simulink model "Porsche930Turbo_Model_V0"  (R2025b)
settings: Solver=ode3  StartTime=0.0  StopTime=1800  FixedStep=0.005  MaxStep=0.01  RelTol=1e-3
values from neighbouring files (symbols this model uses):
  a_front = (1 - CoG_front) * wb    (= 1.32912)    [Main.m]
  af = 1.77    [Main.m]
  bsfc = 395    [Main.m]
  cd = 0.39    [Main.m]
  crr = 0.015    [Main.m]
  distance_imola = s_track    [Main.m]
  eta_gb = 0.95    [Main.m]
  gear_numbers = [1, 2, 3, 4]    [Main.m]
  gear_ratios = [2.25, 1.30, 0.89, 0.625]    [Main.m]
  gear_shift_tbl = [1, 2, 3, 4]    [Main.m]
  grade_imola = grade_track    [Main.m]
  kt = 1.65    [Main.m]
  m_eq = mg + (J_wheels / rw^2) + (J_drivetrain * i_avg^2 / rw^2)    [Main.m]
  mg = mc + (mh * np) + mp_hybrid    (= 1492.5)    [Main.m]
  mu_road = 0.9    [Main.m]
  n_ice = 0:dn:nd    [Main.m]
  ne_em = 0:dn:nemax_em    [Main.m]
  nparallel = 2    [Main.m]
  nseries = 96    [Main.m]
  rho_fuel = 0.75    [Main.m]
  ro = 1.204    [Main.m]
  rt = 4.222    [Main.m]
  rw = (dw * 25.4 / 2 + wt * art / 100) * 1e-3    (= 0.31345)    [Main.m]
  t_ice = zeros(size(n_ice))    [Main.m]
  t_roma_san_basilio = [0 1 2 3 4 5 6 7 8 9 10 11 ... (522 elements, 522x1)]    [ECE_EUDC_Artemis_Bologna_Roma_WLTC_EE_bus.mat]
  tau_turbo = 0.6    [Main.m]
  te_em = zeros(size(ne_em))    [Main.m]
  te_em_peak = zeros(size(ne_em))    [Main.m]
  temax_em = 230    [Main.m]
  tmax_ice = 412    [Main.m]
  track_length = 4909    [Main.m]
  v_cutoff_bp = [0, 0.5, 1.4, 50]    [Main.m]
  v_cutoff_tbl = [0, 0,   1,   1 ]    [Main.m]
  v_ref_imola = v_track_ms    [Main.m]
  v_shift_bp = [0, 18, 33, 48]    [Main.m]
  v_shift_bp_EMODE = [0, 5, 22, 35]    [Main.m]
  vkm_roma_san_basilio = [28.8 30.9 32.4 34.2 35.3 35.6 34.8 33.8 32.2 30.5 29.1 27.9 ... (522 elements, 522x1)]    [ECE_EUDC_Artemis_Bologna_Roma_WLTC_EE_bus.mat]
  wb = 2.272    [Main.m]
undefined symbols (not defined in the file or in its folder): SoC_Per
libraries: simulink x58
(part 3 of 5)

== system Porsche930Turbo_Model_V0/Battery Pack/Subsystem/SOC Evalutation ==
  iB [A] : Inport
  SOH [%] : Inport  Port=2
  Battery Efficency [%] : Constant  Value=BattEff  OutDataTypeStr=single
  Compare To Constant : simulink/Logic and Bit Operations/Compare To Constant  relop=>=  const=0  OutDataTypeStr=boolean
  Constant : Constant  OutDataTypeStr=single
  Constant1 : Constant  OutDataTypeStr=single
  Cp(SOH) : Fcn  Expr=u(1)*u(4)^2 + u(2)*u(4) + u(3)
  Cp_coeff : Constant  Value=Cp  OutDataTypeStr=single
  Display{,1..3} (4 alike) : Display
  Divide : Product  Inputs=*/
  Gain : Gain  Gain=100
  Gain1 : Gain  Gain=1/100
  Gain2 : Gain  Gain=1/100
  Gain3 : Gain  Gain=1/100
  Memory : Memory  InitialCondition=InitialSOC
  Mux6 : Mux  Inputs=2
  Product : Product  OutDataTypeStr=single
  Product1 : Product
  Saturation1 : Saturate  UpperLimit=0.999  LowerLimit=0.001
  Saturation2 : Saturate  UpperLimit=0.999  LowerLimit=0.001
  Sum : Sum  Inputs=+-|  OutDataTypeStr=single
  Switch : Switch  Criteria=u2 > Threshold  SaturateOnIntegerOverflow=off  InputSameDT=off
  "[As] -> [Ah]" : Gain  Gain=1/3600
  dt [s] : SampleTimeMath  TsampMathOp=Ts Only
  SOC [%] : Outport
  wires:
  Cp_coeff/1 -> Display2/1, Mux6/1
  Mux6/1 -> Cp(SOH)/1
  Constant/1 -> dt [s]/1
  dt [s]/1 -> Display/1, Product/1
  Cp(SOH)/1 -> Display3/1, Divide/2
  Gain/1 -> Memory/1, Display1/1, SOC [%]/1
  Saturation1/1 -> Sum/1
  Sum/1 -> Saturation2/1
  Memory/1 -> Gain1/1
  Gain1/1 -> Saturation1/1
  iB [A]/1 -> Compare To Constant/1, Product/2
  "[As] -> [Ah]"/1 -> Sum/2
  Divide/1 -> "[As] -> [Ah]"/1
  Product1/1 -> Divide/1
  Product/1 -> Product1/1
  Switch/1 -> Product1/2
  Constant1/1 -> Switch/1
  Compare To Constant/1 -> Switch/2
  Battery Efficency [%]/1 -> Gain2/1
  Gain2/1 -> Switch/3
  SOH [%]/1 -> Gain3/1
  Gain3/1 -> Mux6/2
  Saturation2/1 -> Gain/1

== system Porsche930Turbo_Model_V0/Battery Pack/Subsystem/Thermal Model ==
  PowrLoss(t) [W] : Inport
  TAmb [°C] : Inport  Port=2
  Compare To Constant : simulink/Logic and Bit Operations/Compare To Constant  relop===  const=2  OutDataTypeStr=boolean
  Compare To Constant1 : simulink/Logic and Bit Operations/Compare To Constant  relop===  const=3  OutDataTypeStr=boolean
  Compare To Constant2 : simulink/Logic and Bit Operations/Compare To Constant  relop===  const=1  OutDataTypeStr=boolean
  Constant : Constant  OutDataTypeStr=single
  Constant1 : Constant  Value=R2Therml  OutDataTypeStr=single
  Constant2 : Constant  Value=R1Therml  OutDataTypeStr=single
  Constant3 : Constant  Value=R3Therml  OutDataTypeStr=single
  Constant4 : Constant  Value=C1Thermal  OutDataTypeStr=single
  Constant5 : Constant  Value=C2Thermal  OutDataTypeStr=single
  Delay : Delay  DelayLength=1  InitialConditionSource=Input port
      settings: InputPortMap=u0,p4
  Delay One Step : Delay  DelayLength=1  InitialCondition=25
  Display Temp : Constant  Value=TRoom  OutDataTypeStr=single
  Merge : Merge  Inputs=3
  Mux : Mux  Inputs=5
  Reference : Constant  Value=ThermReff  OutDataTypeStr=single
  Subsystem : Subsystem
  Subsystem1 : Subsystem
  Subsystem2 : Subsystem
  Sum : Sum  Inputs=|+-
  Switch1 : Switch  Criteria=u2 > Threshold  Threshold=0.5  SaturateOnIntegerOverflow=off  InputSameDT=off
  T_amb : Constant  Value=25
  Thermal Model Selector : Constant  Value=ThermalModelType  OutDataTypeStr=single
  air cooling : MATLAB Function  TreatAsAtomicUnit=on
  dt [s] : SampleTimeMath  TsampMathOp=Ts Only
  CellT [°C] : Outport
  wires:
  Mux/1 -> Subsystem/3(ModelThermalParam), Subsystem1/3(ModelThermalParam)
  Constant2/1 -> Mux/1
  Constant1/1 -> Mux/2
  Constant3/1 -> Mux/3
  Constant4/1 -> Mux/4
  Constant5/1 -> Mux/5
  dt [s]/1 -> Subsystem/4(dt), Subsystem1/4(dt)
  Constant/1 -> dt [s]/1
  Thermal Model Selector/1 -> Compare To Constant/1, Compare To Constant1/1, Compare To Constant2/1
  Compare To Constant/1 -> Subsystem/Enable
  Compare To Constant1/1 -> Subsystem1/Enable
  Subsystem/1(CellT [°C]) -> Merge/2
  Subsystem1/1(CellT [°C]) -> Merge/3
  Merge/1 -> Delay/1
  Delay/1 -> [cellT], CellT [°C]/1
  Display Temp/1 -> Switch1/1
  Reference/1 -> Switch1/2
  TAmb [°C]/1 -> Switch1/3
  Switch1/1 -> Subsystem2/1(TAmb [°C]), Subsystem/1(TAmb [°C]), Delay/2, Subsystem1/1(TAmb [°C])
  Compare To Constant2/1 -> Subsystem2/Enable
  Subsystem2/1(CellT [°C]) -> Merge/1
  [cellT] -> Delay One Step/1
  PowrLoss(t) [W]/1 -> Sum/1
  Sum/1 -> Subsystem1/2(InPower [W]), Subsystem/2(InPower [W])
  [speed] -> air cooling/1(v_car)
  Delay One Step/1 -> air cooling/2(T_cell)
  T_amb/1 -> air cooling/3(T_amb)
  air cooling/1(Q_cool) -> Sum/2

== system Porsche930Turbo_Model_V0/Battery Pack/Subsystem/Vb Evaluation ==
  iB(t) [A] : Inport
  SOC [%] : Inport  Port=2
  SOH [%] : Inport  Port=3
  TCell [°C] : Inport  Port=4
  Gain : Gain  Gain=1/100  OutDataTypeStr=single
  Gain1 : Gain  Gain=1/100
  Product : Product  OutDataTypeStr=single
  Product1 : Product  OutDataTypeStr=single
  R0 : Subsystem
  R0 * iB^2 : Product  OutDataTypeStr=single
  R1 : Subsystem
  Saturation : Saturate  UpperLimit=inf  LowerLimit=0
  Scope : Scope  NumInputPorts=3
      settings: ActiveDisplayYMinimum=-1  ActiveDisplayYMaximum=1  DataLoggingVariableName=ScopeData38
  Sum : Sum  Inputs=+--  OutDataTypeStr=single
  Sum1 : Sum  OutDataTypeStr=single
  VOC : Subsystem
  Vc (t) : Subsystem
  tau1 : Subsystem
  vB(t) [V] : Outport
  PowrLoss(t) [W] : Outport  Port=2
  wires:
  SOC [%]/1 -> Gain/1
  Gain/1 -> tau1/1(SOC [ ]), R1/1(SOC [ ]), R0/1(SOC [ ]), VOC/1(SOC [ ])
  SOH [%]/1 -> Gain1/1
  Gain1/1 -> R0/3(SOH [ ])
  TCell [°C]/1 -> R1/2(TCell [°C]), R0/2(TCell [°C])
  iB(t) [A]/1 -> Saturation/1
  R1/1(R1 [Ohm]) -> Vc (t)/2(R1 [Ohm])
  tau1/1(tau1 [s]) -> Vc (t)/3(tau1 [s])
  VOC/1(VOC [V]) -> Scope/1, Sum/1
  Product/1 -> Scope/2, Sum/2
  R0/1(R0 [Ohm]) -> R0 * iB^2/2, Product/2
  Vc (t)/1(Vc(t) [V]) -> Sum/3, Scope/3
  Sum/1 -> vB(t) [V]/1
  R0 * iB^2/1 -> Sum1/1
  Product1/1 -> R0 * iB^2/1
  Vc (t)/2(PowerLossVc1 [W]) -> Sum1/2
  Sum1/1 -> PowrLoss(t) [W]/1
  Saturation/1 -> Product1/2, Product1/1, Product/1, Vc (t)/1(iB(t) [A])

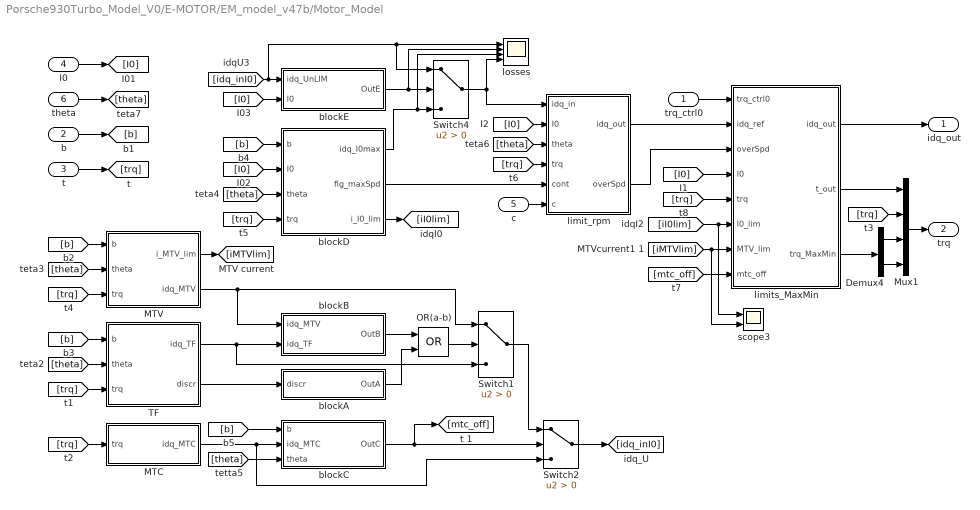
== system Porsche930Turbo_Model_V0/E-MOTOR/EM_model_v47b/Motor_Model ==
  trq_ctrl0 : Inport
  b : Inport  Port=2
  t : Inport  Port=3
  I0 : Inport  Port=4
  c : Inport  Port=5
  theta : Inport  Port=6
  Demux4 : Demux  Outputs=2
  MTC : Subsystem
  MTV : Subsystem
  Mux1 : Mux
  OR(a-b) : Logic  Operator=OR  AllPortsSameDT=off  OutDataTypeStr=boolean
  Switch1 : Switch  Criteria=u2 > Threshold  SaturateOnIntegerOverflow=off  InputSameDT=off
  Switch2 : Switch  Criteria=u2 > Threshold  SaturateOnIntegerOverflow=off  InputSameDT=off
  Switch4 : Switch  Criteria=u2 > Threshold  SaturateOnIntegerOverflow=off  InputSameDT=off
  TF : Subsystem
  blockA : Subsystem
  blockB : Subsystem
  blockC : Subsystem
  blockD : Subsystem
  blockE : Subsystem
  limit_rpm : Subsystem
  limits_MaxMin : Subsystem
  losses : Scope  NumInputPorts=4
      settings: DataLoggingVariableName=ScopeData4  DataLoggingSaveFormat=Array
  scope3 : Scope  NumInputPorts=2
      settings: DataLoggingVariableName=ScopeData8  DataLoggingSaveFormat=Array
  idq_out : Outport
  trq : Outport  Port=2
  wires:
  Mux1/1 -> trq/1
  TF/1(idq_TF) -> Switch1/3, blockB/2(idq_TF)
  OR(a-b)/1 -> Switch1/2
  blockA/1(OutA) -> OR(a-b)/2
  blockB/1(OutB) -> OR(a-b)/1
  Switch1/1 -> Switch2/1
  blockE/1(OutE) -> losses/2, Switch4/2
  blockD/2(flg_maxSpd) -> limit_rpm/5(cont)
  c/1 -> limit_rpm/6(c)
  b/1 -> [b]
  [b] -> MTV/1(b)
  [b] -> TF/1(b)
  [b] -> blockD/1(b)
  [b] -> blockC/1(b)
  [idq_inI0] -> Switch4/1, losses/1, blockE/1(idq_UnLIM)
  I0/1 -> [I0]
  [I0] -> blockD/2(I0)
  [I0] -> blockE/2(I0)
  blockD/1(idq_I0max) -> losses/3, Switch4/3
  TF/2(discr) -> blockA/1(discr)
  theta/1 -> [theta]
  [I0] -> limit_rpm/2(I0)
  [trq] -> Mux1/2
  [trq] -> limit_rpm/4(trq)
  Switch4/1 -> losses/4, limit_rpm/1(idq_in)
  [theta] -> blockC/3(theta)
  [theta] -> TF/2(theta)
  [theta] -> MTV/2(theta)
  [theta] -> blockD/3(theta)
  [theta] -> limit_rpm/3(theta)
  MTV/2(idq_MTV) -> blockB/1(idq_MTV), Switch1/1
  limit_rpm/1(idq_out) -> limits_MaxMin/2(idq_ref)
  limit_rpm/2(overSpd) -> limits_MaxMin/3(overSpd)
  [trq] -> MTV/3(trq)
  [trq] -> blockD/4("trq ")
  t/1 -> [trq]
  Switch2/1 -> [idq_inI0]
  [trq] -> MTC/1(trq)
  [trq] -> TF/3(trq)
  MTC/1(idq_MTC) -> Switch2/3, blockC/2(idq_MTC)
  Demux4/2 -> Mux1/4
  Demux4/1 -> Mux1/3
  trq_ctrl0/1 -> limits_MaxMin/1(trq_ctrl0)
  [I0] -> limits_MaxMin/4(I0)
  MTV/1(i_MTV_lim) -> [iMTVlim]
  blockD/3(i_I0_lim) -> [iI0lim]
  limits_MaxMin/3(trq_MaxMin) -> Demux4/1
  [trq] -> limits_MaxMin/5("trq ")
  limits_MaxMin/2(t_out) -> Mux1/1
  limits_MaxMin/1(idq_out) -> idq_out/1
  blockC/1(OutC) -> Switch2/2, [mtc_off]
  [iMTVlim] -> scope3/2, limits_MaxMin/7(MTV_lim)
  [iI0lim] -> scope3/1, limits_MaxMin/6(I0_lim)
  [mtc_off] -> limits_MaxMin/8(mtc_off)

== system Porsche930Turbo_Model_V0/E-MOTOR/EM_model_v47b/pu_to_real & losses ==
  idq_pu : Inport
  trq_pu : Inport  Port=2
  Vdc : Inport  Port=3
  T0 : Inport  Port=4
  w_m : Inport  Port=5
  rs : Inport  Port=6
  swFreq : Inport  Port=7
  Additional Calc : Subsystem
  Divide : Product  Inputs=**
  Divide1 : Product  Inputs=**
  Divide5 : Product  Inputs=*/
  Manual Switch1 : ManualSwitch
  PWR : Scope
      settings: DataLoggingVariableName=ScopeData3  DataLoggingSaveFormat=Array
  Saturation : Saturate  UpperLimit=1e8  LowerLimit=1
  "[A]" : Constant  Value=In
  eta_calc : Subsystem
  mot+inv losses : Subsystem
  output_mgmt : Subsystem
  pwr_calc : Subsystem
  sc7 : Scope  NumInputPorts=2
      settings: DataLoggingVariableName=ScopeData4  DataLoggingSaveFormat=Array
  trq_derating_TBD : Subsystem
  trq : Outport
  idq : Outport  Port=2
  pwr : Outport  Port=3
  iBat : Outport  Port=4
  eff : Outport  Port=5
  oBus : Outport  Port=6
  wires:
  trq_pu/1 -> trq_derating_TBD/3(trq_pu), Divide1/1
  idq_pu/1 -> trq_derating_TBD/2(idq_pu), Divide/1
  "[A]"/1 -> Divide/2
  T0/1 -> Divide1/2
  Divide/1 -> trq_derating_TBD/1(idq), Manual Switch1/1, sc7/1
  w_m/1 -> [w_m]
  eta_calc/1(eff) -> output_mgmt/7(eff_in)
  Divide5/1 -> output_mgmt/6(iBat_in)
  Vdc/1 -> mot+inv losses/4(Vdc), Divide5/2, Additional Calc/4(Vdc)
  Divide1/1 -> trq_derating_TBD/4(trqIn), mot+inv losses/5(trq), pwr_calc/3(trq), output_mgmt/8(trq_in)
  pwr_calc/1(pwr_vect) -> PWR/1, eta_calc/1(pwr_vect), output_mgmt/4(pwr_vect_in)
  pwr_calc/2(pwrIN) -> Divide5/1
  mot+inv losses/2(losses) -> pwr_calc/1(pwr_loss)
  trq_derating_TBD/1(idq_sat) -> sc7/2, Manual Switch1/2
  swFreq/1 -> Saturation/1
  mot+inv losses/1(other) -> output_mgmt/3(other_in)
  Manual Switch1/1 -> mot+inv losses/1(idq), Additional Calc/3(idq), output_mgmt/2(idq_in)
  [w_m] -> mot+inv losses/3(rad/s)
  [w_m] -> pwr_calc/2(w_m)
  output_mgmt/1(trq) -> trq/1
  output_mgmt/2(idq) -> idq/1
  output_mgmt/3(pwr) -> pwr/1
  output_mgmt/4(iBat) -> iBat/1
  output_mgmt/5(eff) -> eff/1
  [w_m] -> output_mgmt/5(w_m)
  output_mgmt/6(oBus) -> oBus/1
  Saturation/1 -> mot+inv losses/2(swFreq)
  rs/1 -> Additional Calc/1(rs)
  [w_m] -> Additional Calc/2(w_m)
  Additional Calc/1(out) -> output_mgmt/1(add)

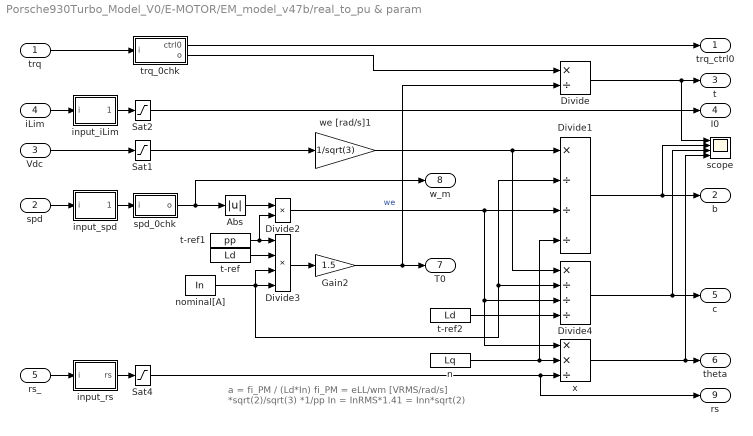
== system Porsche930Turbo_Model_V0/E-MOTOR/EM_model_v47b/real_to_pu & param ==
  note: a = fi_PM / (Ld*In)
      |
      | fi_PM = eLL/wm [VRMS/rad/s] *sqrt(2)/sqrt(3) *1/pp
      |
      | In = InRMS*1.41 = Inn*sqrt(2)
  trq : Inport
  spd : Inport  Port=2
  Vdc : Inport  Port=3
  iLim : Inport  Port=4
  rs_ : Inport  Port=5
  Abs : Abs  SaturateOnIntegerOverflow=off
  Divide : Product  Inputs=*/
  Divide1 : Product  Inputs=*///
  Divide2 : Product  Inputs=**
  Divide3 : Product  Inputs=****
  Divide4 : Product  Inputs=*///
  Gain2 : Gain  Gain=1.5
  Sat1 : Saturate  UpperLimit=3000  LowerLimit=0.1
  Sat2 : Saturate  UpperLimit=33  LowerLimit=0.1
  Sat4 : Saturate  UpperLimit=1  LowerLimit=1e-6
  input_iLim : Subsystem
  input_rs : Subsystem
  input_spd : Subsystem
  "n " : Constant  Value=Lq
  nominal[A] : Constant  Value=In
  scope : Scope  NumInputPorts=4
      settings: DataLoggingVariableName=ScopeData2  DataLoggingSaveFormat=Array
  spd_0chk : Subsystem
  t-ref : Constant  Value=Ld
  t-ref1 : Constant  Value=pp
  t-ref2 : Constant  Value=Ld
  trq_0chk : Subsystem
  we [rad/s]1 : Gain  Gain=1/sqrt(3)
  x : Product  Inputs=**/
  trq_ctrl0 : Outport
  "b " : Outport  Port=2
  t : Outport  Port=3
  I0 : Outport  Port=4
  c : Outport  Port=5
  theta : Outport  Port=6
  T0 : Outport  Port=7
  w_m : Outport  Port=8
  rs : Outport  Port=9
  wires:
  iLim/1 -> input_iLim/1(i)
  Vdc/1 -> Sat1/1
  Divide3/1 -> Gain2/1
  spd/1 -> input_spd/1(i)
  input_iLim/1(iLim) -> Sat2/1
  rs_/1 -> input_rs/1(i)
  input_spd/1(rads) -> spd_0chk/1(i)
  trq/1 -> trq_0chk/1(i)
  trq_0chk/2("o ") -> Divide/1
  x/1 -> scope/4, theta/1
  Sat2/1 -> I0/1
  t-ref2/1 -> Divide4/4
  Sat1/1 -> we [rad/s]1/1
  nominal[A]/1 -> Divide1/2, Divide4/2, Divide3/3, Divide3/4
  Divide2/1 -> x/1, Divide4/3, Divide1/3  "we"
  Gain2/1 -> Divide/2, T0/1
  "n "/1 -> Divide1/4, x/2
  spd_0chk/1(o) -> Abs/1, w_m/1
  input_rs/1(rs) -> Sat4/1
  we [rad/s]1/1 -> Divide4/1, Divide1/1
  Sat4/1 -> rs/1, x/3
  trq_0chk/1(ctrl0) -> trq_ctrl0/1
  t-ref/1 -> Divide3/2
  t-ref1/1 -> Divide2/2, Divide3/1
  Divide/1 -> scope/1, t/1
  Abs/1 -> Divide2/1
  Divide1/1 -> "b "/1, scope/2
  Divide4/1 -> c/1, scope/3

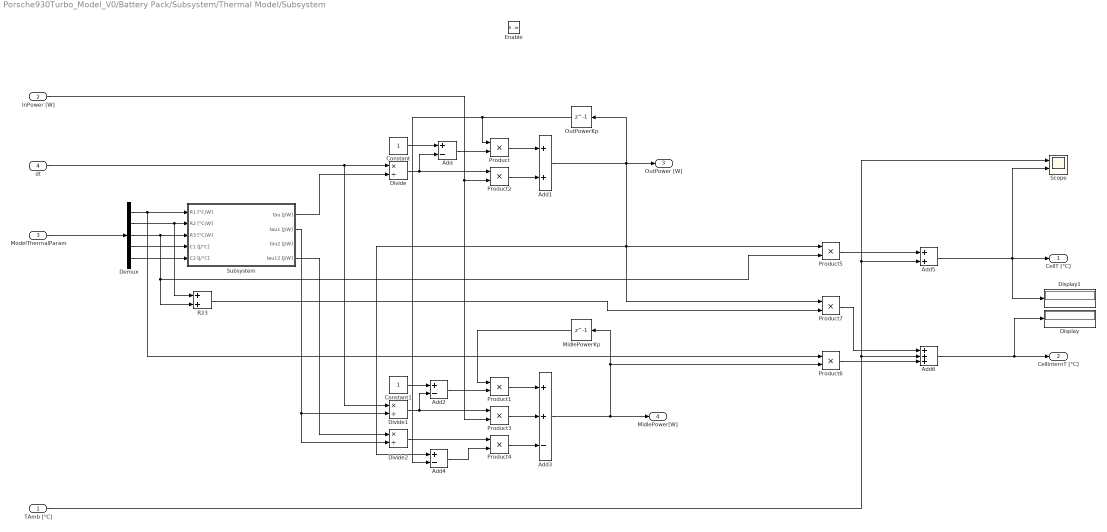
== system Porsche930Turbo_Model_V0/Battery Pack/Subsystem/Thermal Model/Subsystem ==
  TAmb [°C] : Inport
  InPower [W] : Inport  Port=2
  ModelThermalParam : Inport  Port=3
  dt : Inport  Port=4
  Enable : EnablePort
  Add : Sum  Inputs=+-
  Add1 : Sum
  Add2 : Sum  Inputs=+-
  Add3 : Sum  Inputs=++-
  Add4 : Sum  Inputs=+-
  Add5 : Sum
  Add6 : Sum  Inputs=+++
  Constant : Constant  OutDataTypeStr=single
  Constant1 : Constant  OutDataTypeStr=single
  Demux : Demux  Outputs=5
  Display : Display
  Display1 : Display
  Divide : Product  Inputs=*/
  Divide1 : Product  Inputs=*/
  Divide2 : Product  Inputs=*/
  "MidlePowerKp " : Delay  DelayLength=1
  OutPowerKp : Delay  DelayLength=1
  Product{,1..7} (8 alike) : Product  OutDataTypeStr=single
  R23 : Sum
  Scope : Scope  NumInputPorts=2
      settings: DataLoggingSaveFormat=Array
  Subsystem : Subsystem
  CellT [°C] : Outport
  CellInternT [°C] : Outport  Port=2
  OutPower [W] : Outport  Port=3
  MidlePower[W] : Outport  Port=4
  wires:
  Add6/1 -> Display/1, CellInternT [°C]/1
  Product6/1 -> Add6/3
  Product3/1 -> Add3/2
  Divide/1 -> Product2/1, Add/2
  Product5/1 -> Add5/1
  Subsystem/4(tau12 [J/W]) -> Divide2/1
  Add4/1 -> Product4/2
  Product4/1 -> Add3/3
  Add2/1 -> Product1/2
  Subsystem/1(tau [J/W]) -> Divide/2
  Product1/1 -> Add3/1
  Product/1 -> Add1/1
  Constant/1 -> Add/1
  InPower [W]/1 -> Product3/2, Product2/2
  Demux/2 -> R23/1, Subsystem/2(R2 [°C/W])
  dt/1 -> Divide1/1, Divide/1
  TAmb [°C]/1 -> Scope/1, Add5/2, Add6/2
  Demux/3 -> R23/2, Product5/2, Subsystem/3(R3 [°C/W])
  Constant1/1 -> Add2/1
  R23/1 -> Product7/2
  Divide1/1 -> Product3/1, Add2/2
  Divide2/1 -> Product4/1
  Product7/1 -> Add6/1
  Add1/1 -> OutPowerKp/1, Product7/1, Product5/1, Add4/1, OutPower [W]/1
  OutPowerKp/1 -> Add4/2, Product/1
  Demux/5 -> Subsystem/5(C2 [J/°C])
  ModelThermalParam/1 -> Demux/1
  Add/1 -> Product/2
  Demux/4 -> Subsystem/4(C1 [J/°C])
  Subsystem/2(tau1 [J/W]) -> Divide2/2, Divide1/2
  "MidlePowerKp "/1 -> Product1/1
  Product2/1 -> Add1/2
  Demux/1 -> Subsystem/1(R1 [°C/W]), Product6/1
  Add3/1 -> "MidlePowerKp "/1, Product6/2, MidlePower[W]/1
  Add5/1 -> Display1/1, Scope/2, CellT [°C]/1

== system Porsche930Turbo_Model_V0/Battery Pack/Subsystem/Thermal Model/Subsystem1 ==
  TAmb [°C] : Inport
  InPower [W] : Inport  Port=2
  ModelThermalParam : Inport  Port=3
  dt : Inport  Port=4
  Enable : EnablePort
  Add : Sum  Inputs=+-
  Add1 : Sum
  Add5 : Sum
  Constant : Constant  OutDataTypeStr=single
  Demux : Demux  Outputs=5
  Display1 : Display
  Divide : Product  Inputs=*/
  OutPowerKp : Delay  DelayLength=1
  Product : Product  OutDataTypeStr=single
  Product2 : Product  OutDataTypeStr=single
  Product5 : Product  OutDataTypeStr=single
  Scope : Scope  NumInputPorts=2
      settings: DataLoggingSaveFormat=Array
  Subsystem : Subsystem
  Terminator : Terminator
  Terminator1 : Terminator
  CellT [°C] : Outport
  OutPower [W] : Outport  Port=2
  wires:
  Demux/1 -> Subsystem/1(R1 [°C/W])
  Demux/3 -> Product5/2, Subsystem/2(R3 [°C/W])
  dt/1 -> Divide/1
  Constant/1 -> Add/1
  Add5/1 -> Scope/2, CellT [°C]/1, Display1/1
  ModelThermalParam/1 -> Demux/1
  Divide/1 -> Product2/1, Add/2
  TAmb [°C]/1 -> Add5/1, Scope/1
  OutPowerKp/1 -> Product/1
  Product2/1 -> Add1/2
  Add1/1 -> OutPowerKp/1, OutPower [W]/1, Product5/1
  Product/1 -> Add1/1
  Subsystem/1(tau [J/W]) -> Divide/2
  InPower [W]/1 -> Product2/2
  Demux/4 -> Subsystem/3(C1 [J/°C])
  Add/1 -> Product/2
  Demux/2 -> Terminator/1
  Demux/5 -> Terminator1/1
  Product5/1 -> Add5/2

== system Porsche930Turbo_Model_V0/Battery Pack/Subsystem/Thermal Model/Subsystem2 ==
  TAmb [°C] : Inport
  Enable : EnablePort
  CellT [°C] : Outport
  wires:
  TAmb [°C]/1 -> CellT [°C]/1

== system Porsche930Turbo_Model_V0/Battery Pack/Subsystem/Vb Evaluation/R0 ==
  SOC [ ] : Inport
  TCell [°C] : Inport  Port=2
  SOH [ ] : Inport  Port=3
  Display{3..8} (6 alike) : Display
  Mux1 : Mux  Inputs=2
  Mux2 : Mux  Inputs=2
  Mux3 : Mux  Inputs=2
  Product : Product  Inputs=3
  R0 (SOC) : Fcn  Expr=u(1)*u(8)^u(2) + u(3)*log(u(8)) + u(4)*u(8)^3 + u(5)*u(8)^2 +u(6)*u(8) +u(7)
  R0 (SOH) : Fcn  Expr=u(1)*u(4)^2 + u(2)*u(4) + u(3)
  R0 (T) : Fcn  Expr=(u(1)*u(6)^4 + u(2)*u(6)^3 + u(3)*u(6)^2 + u(4)*u(6) + u(5))
  R0SOH_coeff : Constant  Value=R0SOH  OutDataTypeStr=single
  R0T_coeff : Constant  Value=R0T  OutDataTypeStr=single
  R0_coeff : Constant  Value=R0  OutDataTypeStr=single
  R0 [Ohm] : Outport
  wires:
  R0 (SOH)/1 -> Display8/1, Product/3
  R0_coeff/1 -> Mux1/1
  R0SOH_coeff/1 -> Mux3/1
  R0 (SOC)/1 -> Product/1, Display4/1
  Mux3/1 -> R0 (SOH)/1, Display7/1
  Mux2/1 -> R0 (T)/1, Display5/1
  R0T_coeff/1 -> Mux2/1
  Mux1/1 -> Display3/1, R0 (SOC)/1
  Product/1 -> R0 [Ohm]/1
  R0 (T)/1 -> Display6/1, Product/2
  SOC [ ]/1 -> Mux1/2
  TCell [°C]/1 -> Mux2/2
  SOH [ ]/1 -> Mux3/2

== system Porsche930Turbo_Model_V0/Battery Pack/Subsystem/Vb Evaluation/R1 ==
  SOC [ ] : Inport
  TCell [°C] : Inport  Port=2
  Display{9..12} (4 alike) : Display
  Mux4 : Mux  Inputs=2
  Mux5 : Mux  Inputs=2
  Product : Product
  R1 (SOC) : Fcn  Expr=u(1)*u(8)^u(2) + u(3)*log(u(8)) + u(4)*u(8)^3 + u(5)*u(8)^2 +u(6)*u(8) +u(7)
  R1 (T) : Fcn  Expr=(u(1)*u(6)^4 + u(2)*u(6)^3 + u(3)*u(6)^2 + u(4)*u(6) + u(5))
  R1T_coeff : Constant  Value=R1T  OutDataTypeStr=single
  R1_coeff : Constant  Value=R1  OutDataTypeStr=single
  R1 [Ohm] : Outport
  wires:
  Product/1 -> R1 [Ohm]/1
  R1_coeff/1 -> Mux4/1
  R1 (T)/1 -> Display11/1, Product/2
  R1T_coeff/1 -> Mux5/1
  Mux5/1 -> Display10/1, R1 (T)/1
  Mux4/1 -> R1 (SOC)/1, Display9/1
  R1 (SOC)/1 -> Display12/1, Product/1
  TCell [°C]/1 -> Mux5/2
  SOC [ ]/1 -> Mux4/2

== system Porsche930Turbo_Model_V0/Battery Pack/Subsystem/Vb Evaluation/VOC ==
  SOC [ ] : Inport
  Mux : Mux  Inputs=2
  Scope : Scope  NumInputPorts=2
      settings: ActiveDisplayYMinimum=4.0989097952842712  ActiveDisplayYMaximum=4.4228735566139221  DataLoggingVariableName=ScopeData41
  VOC(SOC) : Fcn  Expr=u(1) + u(2)*u(7)+u(3)*u(7)^2+ u(4)/u(7) + u(5)*log(u(7)) + u(6)*log(1-u(7))
  Voc Coeff : Constant  Value=voc  OutDataTypeStr=single
  XY Graph : Record  NumPorts=2.0  FileSettingsInternal="{\"entries\":[{\"content\":{\"excelSettings\":{\"content\":{},\"type\":\"Streamout.ExcelSettings\"},\"parquetSettings\":{\"content\":{},\"type\":\"Streamout.ParquetSettings\"}},\"type\":\"Streamout.FileSettingStorage\",\"uuid\":\"\"}],\"packageUris\":[\"http:\\/\\/schema.mathworks.com\\/mf0\\/streamout_blocks\\/R2020a\"],\"version\":\"1.0\"}"  FrameSettings=[0, 0]  Layout=[1 1]  SignalsInternal="{\"entries\":[{\"content\":{\"signals\":[{\"content\":{\"blockPath\":[],\"dimensions\":[1],\"domain\":\"\",\"lineColor\":\"#edb120\",\"lineWidth\":2,\"port\":1,\"sid\":[\"\"],\"signalID\":1,\"signalName\":\"VOC(SOC)\"},\"type\":\"RecordBlkView.Signal\",\"uuid\":\"\"},{\"content\":{\"blockPath\":[],\"dimensions\":[1],\"domain\":\"\",\"lineColor\":\"#7e2f8e\",\"lineWidth\":2,\"port\":2,\"sid\":[\"\"],\"signalID\":2,\"signalName\":\"SOC [ ]\"},\"type\":\"RecordBlkView.Signal\",\"uuid\":\"\"}]},\"type\":\"RecordBlkView.InputSignals\",\"uuid\":\"\"}],\"packageUris\":[\"http:\\/\\/schema.mathworks.com\\/mf0\\/streamout_blocks\\/R2020a\"],\"version\":\"1.0\"}"  VisualizationBindings="{\"xyplotplugin\":{\"info\":[{\"series\":[],\"subplotID\":1}]}}"  CompatibilityTag=XY
  VOC [V] : Outport
  wires:
  Mux/1 -> Scope/2, VOC(SOC)/1
  SOC [ ]/1 -> XY Graph/2, Mux/2
  Voc Coeff/1 -> Mux/1
  VOC(SOC)/1 -> XY Graph/1, Scope/1, VOC [V]/1

== system Porsche930Turbo_Model_V0/Battery Pack/Subsystem/Vb Evaluation/Vc (t) ==
  iB(t) [A] : Inport
  R1 [Ohm] : Inport  Port=2
  tau1 [s] : Inport  Port=3
  Add : Sum  Inputs=+-  OutDataTypeStr=single  AccumDataTypeStr=single
  Add1 : Sum  OutDataTypeStr=single  AccumDataTypeStr=single
  Constant : Constant  OutDataTypeStr=single
  Constant1 : Constant  OutDataTypeStr=single
  Divide : Product  Inputs=*/  OutDataTypeStr=single
  Divide1 : Product  Inputs=*/  OutDataTypeStr=single
  Memory : Memory
  Product : Product
  Product1 : Product  Inputs=3  OutDataTypeStr=single
  Product2 : Product  OutDataTypeStr=single
  dt [s] : SampleTimeMath  TsampMathOp=Ts Only
  Vc(t) [V] : Outport
  PowerLossVc1 [W] : Outport  Port=2
  wires:
  Divide/1 -> Product1/1, Add/2
  Product/1 -> Add1/1
  Add/1 -> Product/2
  Constant1/1 -> Add/1
  Memory/1 -> Product/1
  Add1/1 -> Vc(t) [V]/1, Product2/2, Product2/1, Memory/1
  Product1/1 -> Add1/2
  R1 [Ohm]/1 -> Divide1/2, Product1/2
  iB(t) [A]/1 -> Product1/3
  tau1 [s]/1 -> Divide/2
  Constant/1 -> dt [s]/1
  dt [s]/1 -> Divide/1
  Product2/1 -> Divide1/1
  Divide1/1 -> PowerLossVc1 [W]/1

== system Porsche930Turbo_Model_V0/Battery Pack/Subsystem/Vb Evaluation/tau1 ==
  SOC [ ] : Inport
  Display15 : Display
  Display16 : Display
  Mux7 : Mux  Inputs=2
  tau1(SOC) : Fcn  Expr=u(1)*u(5)^3 + u(2)*u(5)^2 + u(3)*u(5) + u(4)
  tau1_coeff : Constant  Value=tau1  OutDataTypeStr=single
  tau1 [s] : Outport
  wires:
  SOC [ ]/1 -> Mux7/2
  Mux7/1 -> tau1(SOC)/1, Display15/1
  tau1_coeff/1 -> Mux7/1
  tau1(SOC)/1 -> tau1 [s]/1, Display16/1

== system Porsche930Turbo_Model_V0/E-MOTOR/EM_model_v47b/Motor_Model/MTC ==
  trq : Inport
  " solver_MTC" : MATLAB Function  TreatAsAtomicUnit=on
  Mux4 : Mux  Inputs=2
  a : Constant  Value=a
  "r " : Constant  Value=r
  r 1 : Constant  Value=r1
  sc2 : Scope  NumInputPorts=2
      settings: DataLoggingSaveFormat=Array
  idq_MTC : Outport
  wires:
  "r "/1 -> " solver_MTC"/2(r)
  a/1 -> " solver_MTC"/1(a)
  " solver_MTC"/1(id) -> Mux4/1  "id_MTC"
  " solver_MTC"/2(iq) -> Mux4/2  "iq_MTC"
  trq/1 -> " solver_MTC"/4(t)
  Mux4/1 -> idq_MTC/1, sc2/1
  r 1/1 -> " solver_MTC"/3(r1)
  " solver_MTC"/3(discr) -> sc2/2

== system Porsche930Turbo_Model_V0/E-MOTOR/EM_model_v47b/Motor_Model/MTV ==
  b : Inport
  theta : Inport  Port=2
  trq : Inport  Port=3
  Gain : Gain  Gain=-1
  Mux1 : Mux  Inputs=2
  Mux2 : Mux  Inputs=2
  Mux3 : Mux  Inputs=2
  "a " : Constant  Value=a
  "r " : Constant  Value=r
  r 1 : Constant  Value=r1
  sc2 : Scope  NumInputPorts=2
      settings: DataLoggingVariableName=ScopeData3  DataLoggingSaveFormat=Array
  solver_MTV_neg : MATLAB Function  TreatAsAtomicUnit=on
  solver_MTV_pos : MATLAB Function  TreatAsAtomicUnit=on
  i_MTV_lim : Outport
  idq_MTV : Outport  Port=2
  wires:
  b/1 -> solver_MTV_pos/4(b), solver_MTV_neg/4(b)
  "a "/1 -> solver_MTV_neg/1(a), solver_MTV_pos/1(a)
  "r "/1 -> solver_MTV_neg/2(r), solver_MTV_pos/2(r)
  theta/1 -> solver_MTV_pos/5(theta), solver_MTV_neg/5(theta)
  solver_MTV_pos/1(id) -> Mux1/1  "id_MTV"
  solver_MTV_pos/2(iq) -> Mux1/2  "iq_MTV"
  trq/1 -> solver_MTV_pos/6(t), Gain/1
  Gain/1 -> solver_MTV_neg/6(t)
  Mux1/1 -> idq_MTV/1, sc2/1, Mux3/1
  Mux2/1 -> sc2/2, Mux3/2
  solver_MTV_neg/2(iq) -> Mux2/2  "iq_MTV"
  solver_MTV_neg/1(id) -> Mux2/1  "id_MTV"
  r 1/1 -> solver_MTV_pos/3(r1), solver_MTV_neg/3(r1)
  Mux3/1 -> i_MTV_lim/1

== system Porsche930Turbo_Model_V0/E-MOTOR/EM_model_v47b/Motor_Model/TF ==
  b : Inport
  theta : Inport  Port=2
  trq : Inport  Port=3
  " solver_TF" : MATLAB Function  TreatAsAtomicUnit=on
  Mux3 : Mux  Inputs=2
  a : Constant  Value=a
  "r " : Constant  Value=r
  r 1 : Constant  Value=r1
  sc2 : Scope  NumInputPorts=2
      settings: DataLoggingVariableName=ScopeData2  DataLoggingSaveFormat=Array
  idq_TF : Outport
  discr : Outport  Port=2
  wires:
  " solver_TF"/1(id) -> Mux3/1  "id_TF"
  " solver_TF"/2(iq) -> Mux3/2  "iq_TF"
  a/1 -> " solver_TF"/1(a)
  "r "/1 -> " solver_TF"/2(r)
  " solver_TF"/3(discr) -> sc2/2, discr/1
  Mux3/1 -> sc2/1, idq_TF/1
  b/1 -> " solver_TF"/4(b)
  trq/1 -> " solver_TF"/5(t)
  theta/1 -> " solver_TF"/6(theta)
  r 1/1 -> " solver_TF"/3(r1)

== system Porsche930Turbo_Model_V0/E-MOTOR/EM_model_v47b/Motor_Model/blockA ==
  discr : Inport
  Comp2Const : simulink/Logic and Bit Operations/Compare To Constant  relop=<=  const=0  OutDataTypeStr=boolean
  OutA : Outport
  wires:
  Comp2Const/1 -> OutA/1
  discr/1 -> Comp2Const/1

== system Porsche930Turbo_Model_V0/E-MOTOR/EM_model_v47b/Motor_Model/blockB ==
  idq_MTV : Inport
  idq_TF : Inport  Port=2
  Comp2Const : simulink/Logic and Bit Operations/Compare To Constant  relop=~=  const=0  OutDataTypeStr=boolean
  Logical Operator1 : Logic  AllPortsSameDT=off  OutDataTypeStr=boolean
  Relational Operator : RelationalOperator  Operator=<=  OutDataTypeStr=boolean  InputSameDT=off
  module MTV : Subsystem
      mask Display: disp('DQmod')
  module TF : Subsystem
      mask Display: disp('DQmod')
  slct_id : Selector  InputPortWidth=2  IndexOptions=Index vector (dialog)  Indices=1  OutputSizes=1
  OutB : Outport
  wires:
  idq_MTV/1 -> module MTV/1(i), slct_id/1
  idq_TF/1 -> module TF/1(i)
  module MTV/1(mod) -> Relational Operator/1
  module TF/1(mod) -> Relational Operator/2
  slct_id/1 -> Comp2Const/1
  Comp2Const/1 -> Logical Operator1/2
  Relational Operator/1 -> Logical Operator1/1
  Logical Operator1/1 -> OutB/1

== system Porsche930Turbo_Model_V0/E-MOTOR/EM_model_v47b/Motor_Model/blockC ==
  note: bMTC
  b : Inport
  idq_MTC : Inport  Port=2
  theta : Inport  Port=3
  0chk : Subsystem
      mask Display: disp('0chk')
  Add : Sum  Inputs=+-
  Add2 : Sum
  Add3 : Sum  Inputs=+++
  Constant3 : Constant
  Constant4 : Constant  Value=a
  Constant5 : Constant  Value=r
  Demux1 : Demux  Outputs=2
  Product{4,6..10} (6 alike) : Product
  Product2 : Product  Inputs=*/
  Relational Operator1 : RelationalOperator  Operator=<=  OutDataTypeStr=boolean  InputSameDT=off
  Sqrt : Sqrt
  losses2 : Scope  NumInputPorts=2
      settings: DataLoggingVariableName=ScopeData6  DataLoggingSaveFormat=Array
  OutC : Outport
  wires:
  Demux1/2 -> Add/2, Product6/1  "iq_MTC"
  Demux1/1 -> Product8/1, Product4/1  "id_MTC"
  b/1 -> Relational Operator1/1
  theta/1 -> 0chk/1(i)
  idq_MTC/1 -> Demux1/1
  Constant3/1 -> Product2/1
  0chk/1(o) -> Product2/2
  Product2/1 -> Product4/2, Product6/2
  Product4/1 -> Add/1
  Add/1 -> Product7/2, Product7/1
  Product7/1 -> Add2/1
  Product9/1 -> Add3/3
  Constant4/1 -> Product9/2
  Constant5/1 -> Product9/1, Product8/2
  Add3/1 -> Product10/2, Product10/1
  Product10/1 -> Add2/2
  Add2/1 -> Sqrt/1
  Sqrt/1 -> losses2/1, Relational Operator1/2
  Product6/1 -> Add3/1
  Product8/1 -> Add3/2
  Relational Operator1/1 -> losses2/2, OutC/1

== system Porsche930Turbo_Model_V0/E-MOTOR/EM_model_v47b/Motor_Model/blockD ==
  b : Inport
  I0 : Inport  Port=2
  theta : Inport  Port=3
  "trq " : Inport  Port=4
  Mux4 : Mux  Inputs=2
  Switch2 : Switch  Criteria=u2 > Threshold  SaturateOnIntegerOverflow=off  InputSameDT=off
  Switch5 : Switch  Criteria=u2 > Threshold  SaturateOnIntegerOverflow=off  InputSameDT=off
  id1 : Selector  InputPortWidth=2  IndexOptions=Index vector (dialog)  Indices=1  OutputSizes=1
  id2 : Selector  InputPortWidth=2  IndexOptions=Index vector (dialog)  Indices=1  OutputSizes=1
  id3 : Selector  InputPortWidth=2  IndexOptions=Index vector (dialog)  Indices=1  OutputSizes=1
  idq_max_MTC-I0 : Subsystem
  idq_max_MTV-I0 : Subsystem
  iso controller : Subsystem
  scope : Scope  NumInputPorts=2
      settings: DataLoggingVariableName=ScopeData4  DataLoggingSaveFormat=Array
  scope1 : Scope  NumInputPorts=2
      settings: DataLoggingVariableName=ScopeData3  DataLoggingSaveFormat=Array
  scope2 : Scope  NumInputPorts=2
      settings: DataLoggingVariableName=ScopeData10  DataLoggingSaveFormat=Array
  idq_I0max : Outport
  flg_maxSpd : Outport  Port=2
  i_I0_lim : Outport  Port=3
  wires:
  idq_max_MTV-I0/2(idq_mtvMaxPos) -> id1/1, scope1/1, Switch2/1, scope/1
  Switch2/1 -> Mux4/1, scope2/1, idq_I0max/1
  idq_max_MTV-I0/1(flg_maxSpd) -> flg_maxSpd/1
  iso controller/1(cont_pos) -> Switch2/2
  b/1 -> idq_max_MTV-I0/1(b)
  "trq "/1 -> idq_max_MTC-I0/1(trq), idq_max_MTV-I0/3(trq)
  I0/1 -> idq_max_MTC-I0/2(I0), idq_max_MTV-I0/4(I0)
  theta/1 -> idq_max_MTV-I0/2(theta)
  idq_max_MTC-I0/1(idq_mtcMaxPos) -> id3/1, scope/2, Switch2/3
  iso controller/2(cont_neg) -> Switch5/2
  Switch5/1 -> Mux4/2
  Mux4/1 -> scope2/2, i_I0_lim/1
  idq_max_MTC-I0/2(idq_mtcMaxNeg) -> Switch5/3
  id1/1 -> iso controller/1(id_b_pos)
  id3/1 -> iso controller/3(id_MTC)
  id2/1 -> iso controller/2(id_b_neg)
  idq_max_MTV-I0/3(idq_mtvMaxNeg) -> id2/1, scope1/2, Switch5/1

== system Porsche930Turbo_Model_V0/E-MOTOR/EM_model_v47b/Motor_Model/blockE ==
  idq_UnLIM : Inport
  I0 : Inport  Port=2
  Compare To Constant1 : simulink/Logic and Bit Operations/Compare To Constant  relop=~=  const=0  OutDataTypeStr=boolean
  Logical Operator1 : Logic  AllPortsSameDT=off  OutDataTypeStr=boolean
  Relational Operator : RelationalOperator  Operator=<=  OutDataTypeStr=boolean  InputSameDT=off
  module : Subsystem
  OutE : Outport
  wires:
  idq_UnLIM/1 -> module/1(in)
  module/1(module) -> Compare To Constant1/1, Relational Operator/1
  I0/1 -> Relational Operator/2
  Relational Operator/1 -> Logical Operator1/1
  Logical Operator1/1 -> OutE/1
  Compare To Constant1/1 -> Logical Operator1/2

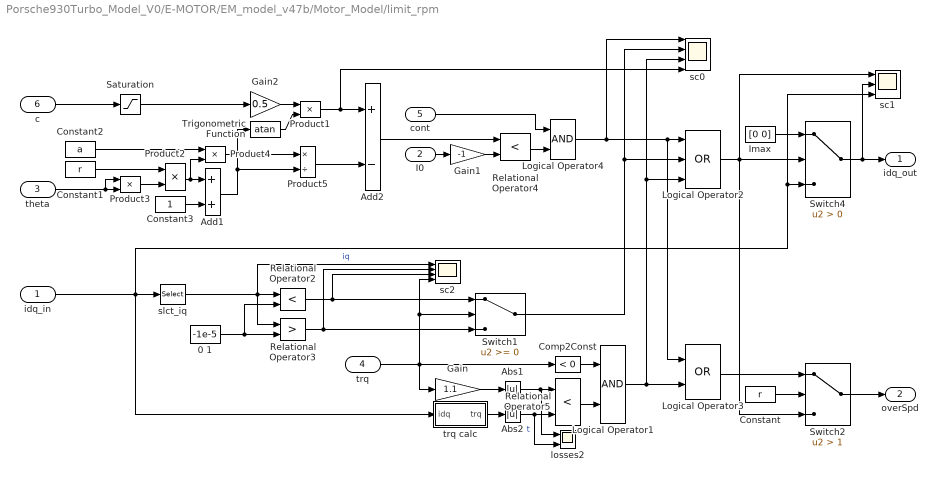
== system Porsche930Turbo_Model_V0/E-MOTOR/EM_model_v47b/Motor_Model/limit_rpm ==
  idq_in : Inport
  I0 : Inport  Port=2
  theta : Inport  Port=3
  trq : Inport  Port=4
  cont : Inport  Port=5
  c : Inport  Port=6
  0 1 : Constant  Value=-1e-5
  Abs1 : Abs  SaturateOnIntegerOverflow=off
  Abs2 : Abs  SaturateOnIntegerOverflow=off
  Add1 : Sum
  Add2 : Sum  Inputs=+-
  Comp2Const : simulink/Logic and Bit Operations/Compare To Constant  relop=<  const=0  OutDataTypeStr=boolean
  Constant : Constant  Value=r
  Constant1 : Constant  Value=r
  Constant2 : Constant  Value=a
  Constant3 : Constant
  Gain : Gain  Gain=1.1
  Gain1 : Gain  Gain=-1
  Gain2 : Gain  Gain=0.5
  Imax : Constant  Value=[0 0]
  Logical Operator1 : Logic  AllPortsSameDT=off  OutDataTypeStr=boolean
  Logical Operator2 : Logic  Operator=OR  Inputs=3  AllPortsSameDT=off  OutDataTypeStr=boolean
  Logical Operator3 : Logic  Operator=OR  AllPortsSameDT=off  OutDataTypeStr=boolean
  Logical Operator4 : Logic  AllPortsSameDT=off  OutDataTypeStr=boolean
  Product{1..4} (4 alike) : Product
  Product5 : Product  Inputs=*/
  Relational Operator2 : RelationalOperator  Operator=<  OutDataTypeStr=boolean  InputSameDT=off
  Relational Operator3 : RelationalOperator  Operator=>  OutDataTypeStr=boolean  InputSameDT=off
  Relational Operator4 : RelationalOperator  Operator=<  OutDataTypeStr=boolean  InputSameDT=off
  Relational Operator5 : RelationalOperator  Operator=<  OutDataTypeStr=boolean  InputSameDT=off
  Saturation : Saturate  UpperLimit=20000  LowerLimit=0
  Switch1 : Switch  SaturateOnIntegerOverflow=off  InputSameDT=off
  Switch2 : Switch  Criteria=u2 > Threshold  Threshold=1  SaturateOnIntegerOverflow=off  InputSameDT=off
  Switch4 : Switch  Criteria=u2 > Threshold  SaturateOnIntegerOverflow=off  InputSameDT=off
  Trigonometric Function : Trigonometry  Operator=atan
  losses2 : Scope  NumInputPorts=2
      settings: DataLoggingVariableName=ScopeData7  DataLoggingSaveFormat=Array
  sc0 : Scope  NumInputPorts=4
      settings: DataLoggingVariableName=ScopeData5  DataLoggingSaveFormat=Array
  sc1 : Scope  NumInputPorts=3
      settings: DataLoggingVariableName=ScopeData3  DataLoggingSaveFormat=Array
  sc2 : Scope  NumInputPorts=4
      settings: DataLoggingVariableName=ScopeData6  DataLoggingSaveFormat=Array
  slct_iq : Selector  InputPortWidth=2  IndexOptions=Index vector (dialog)  Indices=2  OutputSizes=1
  trq calc : Subsystem
  idq_out : Outport
  overSpd : Outport  Port=2
  wires:
  Switch4/1 -> idq_out/1, sc1/2
  Imax/1 -> Switch4/1
  I0/1 -> Gain1/1
  Logical Operator2/1 -> Switch4/2, Switch2/3, sc1/1
  slct_iq/1 -> sc2/1, Relational Operator3/1, Relational Operator2/1  "iq"
  0 1/1 -> Relational Operator2/2, Relational Operator3/2
  Relational Operator2/1 -> sc2/3, Switch1/1
  Switch1/1 -> sc0/2, Logical Operator2/2
  Relational Operator3/1 -> sc2/2, Switch1/3
  Logical Operator1/1 -> sc0/3, Logical Operator2/3, Logical Operator3/2
  Logical Operator4/1 -> sc0/1, Logical Operator2/1, Logical Operator3/1
  Switch2/1 -> overSpd/1
  Logical Operator3/1 -> Switch2/1
  Constant/1 -> Switch2/2
  Add2/1 -> Relational Operator4/1
  Product1/1 -> sc0/4, Add2/1
  Gain1/1 -> Relational Operator4/2
  Relational Operator4/1 -> Logical Operator4/2
  cont/1 -> Logical Operator4/1
  Constant2/1 -> Product4/1
  Trigonometric Function/1 -> Product1/2
  Product5/1 -> Add2/2
  Add1/1 -> Product5/2, Trigonometric Function/1
  Product3/1 -> Product2/2
  Constant3/1 -> Add1/2
  theta/1 -> Product3/1, Product3/2
  Product2/1 -> Product4/2, Add1/1
  Gain2/1 -> Product1/1
  Saturation/1 -> Gain2/1
  Product4/1 -> Product5/1
  Constant1/1 -> Product2/1
  c/1 -> Saturation/1
  trq/1 -> Gain/1, sc2/4, Switch1/2, Comp2Const/1
  Relational Operator5/1 -> Logical Operator1/2
  Comp2Const/1 -> Logical Operator1/1
  Gain/1 -> Abs1/1
  Abs2/1 -> Relational Operator5/2, losses2/2  "t"
  idq_in/1 -> Switch4/3, sc1/3, trq calc/1(idq), slct_iq/1
  Abs1/1 -> losses2/1, Relational Operator5/1
  trq calc/1(trq) -> Abs2/1

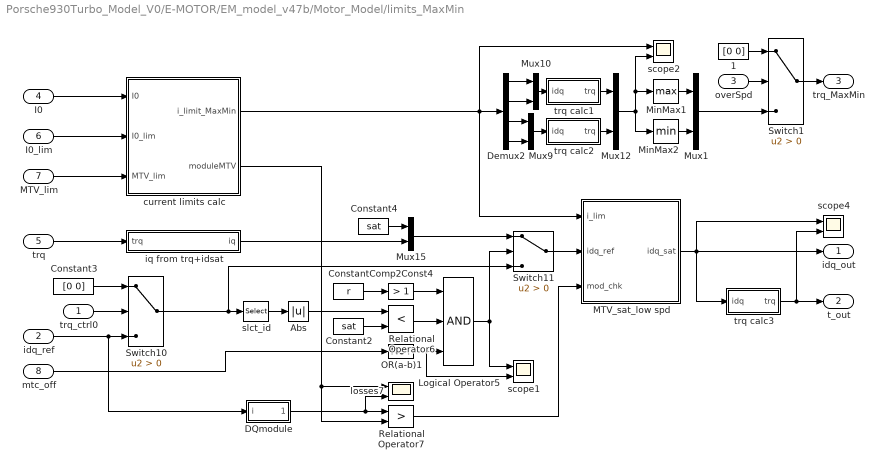
== system Porsche930Turbo_Model_V0/E-MOTOR/EM_model_v47b/Motor_Model/limits_MaxMin ==
  trq_ctrl0 : Inport
  idq_ref : Inport  Port=2
  overSpd : Inport  Port=3
  I0 : Inport  Port=4
  "trq " : Inport  Port=5
  I0_lim : Inport  Port=6
  MTV_lim : Inport  Port=7
  mtc_off : Inport  Port=8
  1 : Constant  Value=[0 0]
  Abs : Abs  SaturateOnIntegerOverflow=off
  Comp2Const4 : simulink/Logic and Bit Operations/Compare To Constant  relop=>  const=1  OutDataTypeStr=boolean
  Constant : Constant  Value=r
  Constant2 : Constant  Value=sat
  Constant3 : Constant  Value=[0 0]
  Constant4 : Constant  Value=sat
  DQmodule : Subsystem
      mask Display: disp('DQmod')
  Demux2 : Demux
  Logical Operator5 : Logic  Inputs=3  AllPortsSameDT=off  OutDataTypeStr=boolean
  MTV_sat_low spd : Subsystem
  MinMax1 : MinMax  Function=max
  MinMax2 : MinMax
  Mux{1,9..10,12,15} (5 alike) : Mux  Inputs=2
  OR(a-b)1 : Logic  Operator=NOT  AllPortsSameDT=off  OutDataTypeStr=boolean
  Relational Operator6 : RelationalOperator  Operator=<  OutDataTypeStr=boolean  InputSameDT=off
  Relational Operator7 : RelationalOperator  Operator=>  OutDataTypeStr=boolean  InputSameDT=off
  Switch1 : Switch  Criteria=u2 > Threshold  SaturateOnIntegerOverflow=off  InputSameDT=off
  Switch10 : Switch  Criteria=u2 > Threshold  SaturateOnIntegerOverflow=off  InputSameDT=off
  Switch11 : Switch  Criteria=u2 > Threshold  SaturateOnIntegerOverflow=off  InputSameDT=off
  current limits calc : Subsystem
  iq from trq+idsat : Subsystem
  losses7 : Scope  NumInputPorts=2
      settings: DataLoggingVariableName=ScopeData20  DataLoggingSaveFormat=Array
  scope1 : Scope  NumInputPorts=2
      settings: DataLoggingVariableName=ScopeData16  DataLoggingSaveFormat=Array
  scope2 : Scope  NumInputPorts=2
      settings: DataLoggingSaveFormat=Array
  scope4 : Scope  NumInputPorts=2
      settings: DataLoggingVariableName=ScopeData19  DataLoggingSaveFormat=Array
  slct_id : Selector  InputPortWidth=2  IndexOptions=Index vector (dialog)  Indices=1  OutputSizes=1
  trq calc1 : Subsystem
  trq calc2 : Subsystem
  trq calc3 : Subsystem
  idq_out : Outport
  t_out : Outport  Port=2
  trq_MaxMin : Outport  Port=3
  wires:
  Demux2/2 -> Mux10/2
  Mux9/1 -> trq calc2/1(idq)
  Demux2/1 -> Mux10/1
  Demux2/3 -> Mux9/1
  Demux2/4 -> Mux9/2
  Mux10/1 -> trq calc1/1(idq)
  trq calc1/1(trq) -> Mux12/1
  trq calc2/1(trq) -> Mux12/2
  Mux12/1 -> MinMax2/1, scope2/2, MinMax1/1
  MinMax1/1 -> Mux1/1
  MinMax2/1 -> Mux1/2
  Comp2Const4/1 -> Logical Operator5/1
  trq_ctrl0/1 -> Switch10/2
  Abs/1 -> Relational Operator6/1
  Switch10/1 -> slct_id/1, Switch11/3
  trq calc3/1(trq) -> t_out/1, scope4/2
  Mux15/1 -> Switch11/1
  "trq "/1 -> iq from trq+idsat/1(trq)
  OR(a-b)1/1 -> Logical Operator5/3, scope1/2
  Constant/1 -> Comp2Const4/1
  slct_id/1 -> Abs/1
  Relational Operator6/1 -> Logical Operator5/2
  Logical Operator5/1 -> Switch11/2, scope1/1
  Constant2/1 -> Relational Operator6/2
  iq from trq+idsat/1(iq) -> Mux15/2
  idq_ref/1 -> DQmodule/1(i), Switch10/3
  Constant3/1 -> Switch10/1
  mtc_off/1 -> OR(a-b)1/1
  Constant4/1 -> Mux15/1
  DQmodule/1(mod) -> Relational Operator7/1, losses7/2
  1/1 -> Switch1/1
  overSpd/1 -> Switch1/2
  Mux1/1 -> Switch1/3
  Switch1/1 -> trq_MaxMin/1
  current limits calc/2(moduleMTV) -> losses7/1, Relational Operator7/2
  current limits calc/1(i_limit_MaxMin) -> scope2/1, MTV_sat_low spd/1(i_lim), Demux2/1
  I0/1 -> current limits calc/1(I0)
  MTV_lim/1 -> current limits calc/3(MTV_lim)
  I0_lim/1 -> current limits calc/2(I0_lim)
  MTV_sat_low spd/1(idq_sat) -> scope4/1, trq calc3/1(idq), idq_out/1
  Switch11/1 -> MTV_sat_low spd/2(idq_ref)
  Relational Operator7/1 -> MTV_sat_low spd/3(mod_chk)

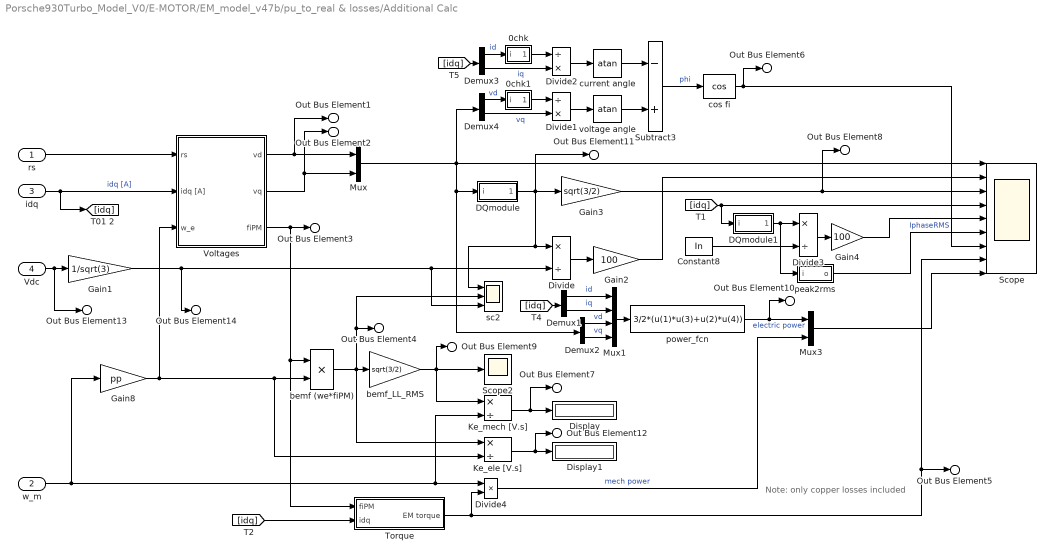
== system Porsche930Turbo_Model_V0/E-MOTOR/EM_model_v47b/pu_to_real & losses/Additional Calc ==
  note: Note: only copper losses included
  rs : Inport
  w_m : Inport  Port=2
  idq : Inport  Port=3
  Vdc : Inport  Port=4
  0chk : Subsystem
      mask Display: disp('0chk')
  0chk1 : Subsystem
      mask Display: disp('0chk')
  Constant8 : Constant  Value=In
  DQmodule : Subsystem
      mask Display: disp('DQmod')
  DQmodule1 : Subsystem
      mask Display: disp('DQmod')
  Demux{1..4} (4 alike) : Demux  Outputs=2
  Display : Display
  Display1 : Display
  Divide : Product  Inputs=*/
  Divide1 : Product  Inputs=/*
  Divide2 : Product  Inputs=/*
  Divide3 : Product  Inputs=*/
  Divide4 : Product  Inputs=**
  Gain1 : Gain  Gain=1/sqrt(3)
  Gain2 : Gain  Gain=100
  Gain3 : Gain  Gain=sqrt(3/2)
  Gain4 : Gain  Gain=100
  Gain8 : Gain  Gain=pp
  Ke_ele [V.s] : Product  Inputs=*/
  Ke_mech [V.s] : Product  Inputs=*/
  Mux : Mux  Inputs=2
  Mux1 : Mux
  Mux3 : Mux  Inputs=2
  Scope : Scope  NumInputPorts=9
      settings: Title=Vd Vq VOLTAGE  DataLoggingSaveFormat=Array
  Scope2 : Scope
      settings: DataLoggingSaveFormat=Array
  Subtract3 : Sum  Inputs=-+
  Torque : Subsystem
  Voltages : Subsystem
  bemf (we*fiPM) : Product
  bemf_LL_RMS : Gain  Gain=sqrt(3/2)
  cos fi : Trigonometry  Operator=cos
  current angle : Trigonometry  Operator=atan
  peak2rms : Subsystem
      mask Display: disp('pk2rms')
  power_fcn : Fcn  Expr=3/2*(u(1)*u(3)+u(2)*u(4))
  sc2 : Scope  NumInputPorts=3
      settings: DataLoggingSaveFormat=Array
  voltage angle : Trigonometry  Operator=atan
  Out Bus Element1 : Outport  PortName=out  Element=vd
  Out Bus Element2 : Outport  PortName=out  Element=vq
  Out Bus Element11 : Outport  PortName=out  Element=v_mod
  Out Bus Element8 : Outport  PortName=out  Element=v_LLrms
  Out Bus Element3 : Outport  PortName=out  Element=f_pm
  Out Bus Element4 : Outport  PortName=out  Element=bemf
  Out Bus Element9 : Outport  PortName=out  Element=bemf_LLrms
  Out Bus Element6 : Outport  PortName=out  Element=cos_phi
  Out Bus Element7 : Outport  PortName=out  Element=Ke_mec
  Out Bus Element12 : Outport  PortName=out  Element=Ke_ele
  Out Bus Element5 : Outport  PortName=out  Element=e_trq
  Out Bus Element10 : Outport  PortName=out  Element=e_pwr
  Out Bus Element13 : Outport  PortName=out  Element=Vdc
  Out Bus Element14 : Outport  PortName=out  Element=Vphase
  wires:
  Vdc/1 -> Out Bus Element13/1, Gain1/1
  Gain1/1 -> Out Bus Element14/1, sc2/3, Divide/2
  DQmodule/1(mod) -> Gain3/1, sc2/1, Divide/1, Out Bus Element11/1
  Divide/1 -> Gain2/1
  Gain2/1 -> Scope/2
  Mux/1 -> DQmodule/1(i), Demux2/1, Demux4/1, Scope/1
  idq/1 -> [idq], Voltages/2(idq [A])  "idq [A]"
  Divide1/1 -> voltage angle/1
  Divide2/1 -> current angle/1
  current angle/1 -> Subtract3/1
  voltage angle/1 -> Subtract3/2
  Subtract3/1 -> cos fi/1  "phi"
  cos fi/1 -> Scope/7, Out Bus Element6/1
  Demux1/1 -> Mux1/1  "id"
  Demux1/2 -> Mux1/2  "iq"
  Mux1/1 -> power_fcn/1
  Gain3/1 -> Out Bus Element8/1, Scope/3
  DQmodule1/1(mod) -> peak2rms/1(i), Divide3/1
  Divide3/1 -> Gain4/1
  Gain4/1 -> Scope/5
  peak2rms/1(o) -> Scope/6  "IphaseRMS"
  Divide4/1 -> Mux3/2  "mech power"
  Mux3/1 -> Scope/9
  power_fcn/1 -> Mux3/1, Out Bus Element10/1  "electric power"
  bemf (we*fiPM)/1 -> sc2/2, Out Bus Element4/1, Ke_ele [V.s]/1, bemf_LL_RMS/1
  bemf_LL_RMS/1 -> Scope2/1, Ke_mech [V.s]/1, Out Bus Element9/1
  Ke_mech [V.s]/1 -> Out Bus Element7/1, Display/1
  [idq] -> Demux1/1
  [idq] -> DQmodule1/1(i), Scope/4
  [idq] -> Demux3/1
  Demux3/1 -> 0chk/1(i)  "id"
  Demux3/2 -> Divide2/2  "iq"
  Constant8/1 -> Divide3/2
  Gain8/1 -> Ke_ele [V.s]/2, bemf (we*fiPM)/2, Voltages/3(w_e)
  Voltages/1(vd) -> Mux/1, Out Bus Element1/1
  Voltages/2(vq) -> Out Bus Element2/1, Mux/2
  Voltages/3(fiPM) -> Out Bus Element3/1, bemf (we*fiPM)/1, Torque/1(fiPM)
  rs/1 -> Voltages/1(rs)
  Torque/1(EM torque) -> Scope/8, Out Bus Element5/1, Divide4/2
  [idq] -> Torque/2(idq)
  Demux2/1 -> Mux1/3  "vd"
  Demux2/2 -> Mux1/4  "vq"
  Demux4/1 -> 0chk1/1(i)  "vd"
  Demux4/2 -> Divide1/2  "vq"
  0chk/1(o) -> Divide2/1
  0chk1/1(o) -> Divide1/1
  w_m/1 -> Gain8/1, Ke_mech [V.s]/2, Divide4/1
  Ke_ele [V.s]/1 -> Display1/1, Out Bus Element12/1

== system Porsche930Turbo_Model_V0/E-MOTOR/EM_model_v47b/pu_to_real & losses/eta_calc ==
  pwr_vect : Inport
  0chk : Subsystem
      mask Display: disp('0chk')
  0chk1 : Subsystem
      mask Display: disp('0chk')
  0chk2 : Subsystem
      mask Display: disp('0chk')
  Demux1 : Demux
  Divide2 : Product  Inputs=*/
  Divide3 : Product  Inputs=*/
  Divide4 : Product  Inputs=/*
  Divide5 : Product  Inputs=/*
  Divide6 : Product  Inputs=*/
  Divide7 : Product  Inputs=/*
  Mux5 : Mux  Inputs=3
  Saturation : Saturate  UpperLimit=1  LowerLimit=0
  Saturation1 : Saturate  UpperLimit=1  LowerLimit=0
  Saturation2 : Saturate  UpperLimit=1  LowerLimit=0
  Sum1 : Sum
  Sum4 : Sum  Inputs=+-
  Switch1 : Switch  SaturateOnIntegerOverflow=off  InputSameDT=off
  Switch2 : Switch  SaturateOnIntegerOverflow=off  InputSameDT=off
  Switch3 : Switch  SaturateOnIntegerOverflow=off  InputSameDT=off
  sc1 : Scope  NumInputPorts=3
      settings: DataLoggingVariableName=ScopeData10  DataLoggingSaveFormat=Array
  sc2 : Scope  NumInputPorts=4
      settings: DataLoggingVariableName=ScopeData9  DataLoggingSaveFormat=Array
  sc7 : Scope  NumInputPorts=3
      settings: DataLoggingSaveFormat=Array
  slct : Selector  InputPortWidth=9  IndexOptions=Index vector (dialog)  Indices=[1 2 4 5]  OutputSizes=1
  eff : Outport
  wires:
  Switch2/1 -> Saturation/1
  Divide4/1 -> Switch2/1
  Saturation/1 -> sc1/1, Mux5/1  "tot"
  Divide3/1 -> Switch2/3
  0chk/1(o) -> sc7/1, Divide3/1, Divide4/1, Divide6/1, Divide7/1  "DC"
  Demux1/4 -> Sum4/2  "inv_loss"
  Switch3/1 -> Saturation2/1
  Saturation1/1 -> sc1/2, Mux5/2  "mot"
  Demux1/3 -> Sum1/2  "mot_loss"
  Switch1/1 -> Saturation1/1
  Saturation2/1 -> sc1/3, Mux5/3  "inv"
  Sum1/1 -> sc2/2, 0chk2/1(i)
  Divide5/1 -> Switch1/1
  Divide2/1 -> Switch1/3
  0chk2/1(o) -> sc7/2, Divide6/2, Switch3/2, Divide7/2, Divide2/1, Divide5/1  "3Ph"
  Demux1/2 -> sc2/4, Sum1/1, 0chk1/1(i)  "pwrOut"
  Divide7/1 -> Switch3/1
  Divide6/1 -> Switch3/3
  0chk1/1(o) -> Divide3/2, Switch2/2, sc7/3, Divide4/2, Divide5/2, Switch1/2, Divide2/2  "Mech"
  Demux1/1 -> Sum4/1, 0chk/1(i), sc2/1  "pwrIn"
  pwr_vect/1 -> slct/1
  slct/1 -> Demux1/1
  Mux5/1 -> eff/1
  Sum4/1 -> sc2/3

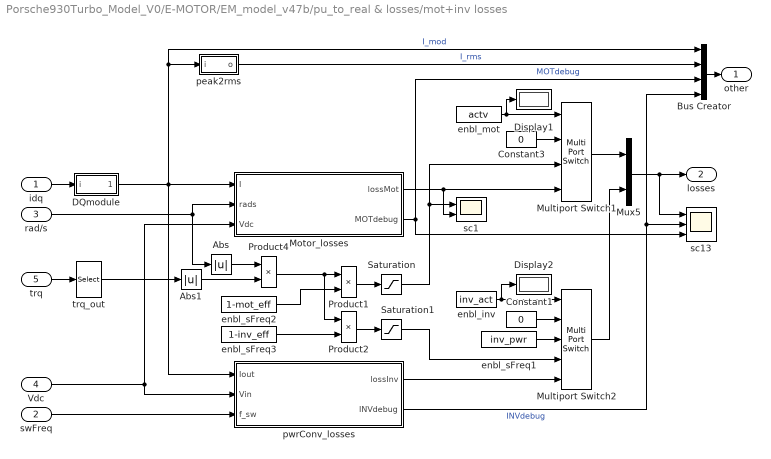
== system Porsche930Turbo_Model_V0/E-MOTOR/EM_model_v47b/pu_to_real & losses/mot+inv losses ==
  idq : Inport
  swFreq : Inport  Port=2
  rad/s : Inport  Port=3
  Vdc : Inport  Port=4
  trq : Inport  Port=5
  Abs : Abs  SaturateOnIntegerOverflow=off
  Abs1 : Abs  SaturateOnIntegerOverflow=off
  Bus Creator : BusCreator  Inputs=4
  Constant1 : Constant  Value=0
  Constant3 : Constant  Value=0
  DQmodule : Subsystem
      mask Display: disp('DQmod')
  Display1 : Display
  Display2 : Display
  Motor_losses : Subsystem
  Multiport Switch1 : MultiPortSwitch  SaturateOnIntegerOverflow=off  InputSameDT=off
  Multiport Switch2 : MultiPortSwitch  Inputs=4  SaturateOnIntegerOverflow=off  InputSameDT=off
  Mux5 : Mux  Inputs=2
  Product1 : Product  Inputs=**
  Product2 : Product  Inputs=**
  Product4 : Product  Inputs=**
  Saturation : Saturate  UpperLimit=1e6  LowerLimit=1
  Saturation1 : Saturate  UpperLimit=1e6  LowerLimit=1
  enbl_inv : Constant  Value=inv_act
  enbl_mot : Constant  Value=actv
  enbl_sFreq1 : Constant  Value=inv_pwr
  enbl_sFreq2 : Constant  Value=1-mot_eff
  enbl_sFreq3 : Constant  Value=1-inv_eff
  peak2rms : Subsystem
      mask Display: disp('pk2rms')
  pwrConv_losses : Subsystem
  sc1 : Scope  NumInputPorts=2
      settings: DataLoggingSaveFormat=Array
  sc13 : Scope  NumInputPorts=3
      settings: DataLoggingVariableName=ScopeData2  DataLoggingSaveFormat=Array
  trq_out : Selector  InputPortWidth=4  IndexOptions=Index vector (dialog)  Indices=1  OutputSizes=1
  other : Outport
  losses : Outport  Port=2
  wires:
  idq/1 -> DQmodule/1(i)
  Multiport Switch1/1 -> Mux5/1
  pwrConv_losses/1(lossInv) -> Multiport Switch2/5
  Multiport Switch2/1 -> Mux5/2
  Mux5/1 -> sc13/1, losses/1
  Vdc/1 -> Motor_losses/3(Vdc), pwrConv_losses/2(Vin)
  DQmodule/1(mod) -> peak2rms/1(i), Bus Creator/1, pwrConv_losses/1(Iout), Motor_losses/1(I)  "I_mod"
  peak2rms/1(o) -> Bus Creator/2  "I_rms"
  enbl_inv/1 -> Display2/1, Multiport Switch2/1
  Constant1/1 -> Multiport Switch2/2
  enbl_sFreq1/1 -> Multiport Switch2/3
  pwrConv_losses/2(INVdebug) -> Bus Creator/4, sc13/2  "INVdebug"
  rad/s/1 -> Abs/1, Motor_losses/2(rads)
  Motor_losses/1(lossMot) -> sc1/2, Multiport Switch1/4
  trq/1 -> trq_out/1
  trq_out/1 -> Abs1/1
  enbl_mot/1 -> Display1/1, Multiport Switch1/1
  Constant3/1 -> Multiport Switch1/2
  Product4/1 -> Product2/1, Product1/1
  Abs/1 -> Product4/1
  Abs1/1 -> Product4/2
  Saturation/1 -> Multiport Switch1/3, sc1/1
  Bus Creator/1 -> other/1
  Product1/1 -> Saturation/1
  enbl_sFreq2/1 -> Product1/2
  Product2/1 -> Saturation1/1
  enbl_sFreq3/1 -> Product2/2
  Saturation1/1 -> Multiport Switch2/4
  Motor_losses/2(MOTdebug) -> sc13/3, Bus Creator/3  "MOTdebug"
  swFreq/1 -> pwrConv_losses/3(f_sw)
